simulink model "voyager1"  (R2025b)
settings: Solver=VariableStepAuto  StartTime=0.0  StopTime=2  RelTol=1e-3
values from neighbouring files (symbols this model uses):
  h = h/sum(h)    [voyager.m]
libraries: simulink x1
settings Model: Creator=HP  LastModifiedBy=HP

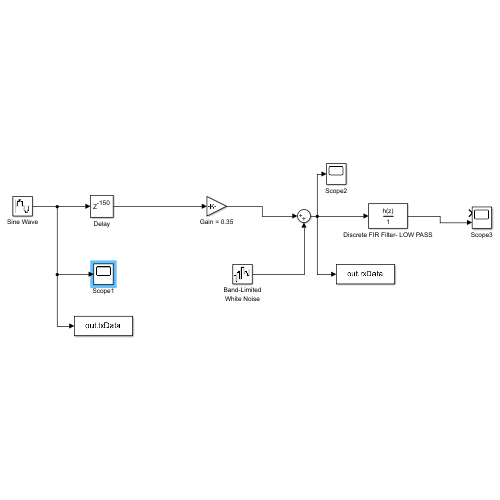
[thumbnail: Simulink's stored preview of the top-level diagram]
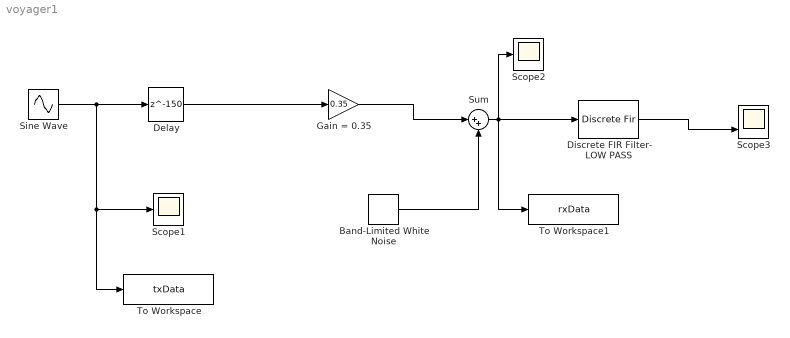
== system voyager1 ==
  Band-Limited White Noise : simulink/Sources/Band-Limited White Noise  Cov=[0.1]  Ts=0.001  seed=[23341]
  Delay : Delay  DelayLength=150
  Discrete FIR Filter- LOW PASS : DiscreteFir  Coefficients=h
  Gain = 0.35 : Gain  Gain=0.35
  Scope1 : Scope
      settings: ActiveDisplayYMinimum=-20.630645054143315  ActiveDisplayYMaximum=13.576142108182971  DataLoggingVariableName=ScopeData2
  Scope2 : Scope
      settings: ActiveDisplayYMinimum=-45.255454716979827  ActiveDisplayYMaximum=48.46740218507275
  Scope3 : Scope  NumInputPorts=2
      settings: ActiveDisplayYMinimum=-16.364884244140956  ActiveDisplayYMaximum=14.529916808028037
  Sine Wave : Sin  Frequency=125.6637  SampleTime=0.001
  Sum : Sum  Inputs=|++
  To Workspace : ToWorkspace  VariableName=txData  SaveFormat=Timeseries  SampleTime=-1
  To Workspace1 : ToWorkspace  VariableName=rxData  SaveFormat=Timeseries  SampleTime=-1
  wires:
  Gain = 0.35/1 -> Sum/1
  Band-Limited White Noise/1 -> Sum/2
  Sum/1 -> To Workspace1/1, Discrete FIR Filter- LOW PASS/1, Scope2/1
  Discrete FIR Filter- LOW PASS/1 -> Scope3/2
  Delay/1 -> Gain = 0.35/1
  Sine Wave/1 -> Delay/1, To Workspace/1, Scope1/1
